simulink model "Commander_Stabilizer_QDrone"  (R2021b)
settings: Solver=ode1  StartTime=0.0  StopTime=inf  FixedStep=0.001  RelTol=1e-3  EnableMultiTasking=on
InitFcn:
  | set_param(gcs, 'ZoomFactor','FitSystem')
model workspace (MAT data in the model file):
  target_system = 1
undefined symbols (not defined in the file): HIL, qc_get_step_size
libraries: quarc_library x49, simulink x23, simulink_extras x5
(part 3 of 3)

== system Commander_Stabilizer_QDrone/PHYSICAL PLANT w// LINEAR THRUST/Sensor Failure Monitoring/Sensor Failure (Accelerometer) ==
  note: Check for flat-line ZERO Accelerometer data (no data)
  Sensor Input : Inport
  Clock : Clock
  Compare To Constant : simulink/Logic and Bit Operations/Compare To Constant  relop=>=  const=1  OutDataTypeStr=boolean
  Demux1 : Demux  Outputs=3
  Logical Operator : Logic  Operator=OR  Inputs=3  AllPortsSameDT=off  OutDataTypeStr=boolean
  Logical Operator1 : Logic  AllPortsSameDT=off  OutDataTypeStr=boolean
  Terminator1 : Terminator
  Terminator3 : Terminator
  Terminator4 : Terminator
  Threshold : quarc_library/Discontinuities/Threshold  operator===  param_src=Specify via dialog  threshold=0  duration=1
      settings: SourceProductName=The database C:\Users\user\AppData\Roaming\MathWorks\MATLAB\R2017a\slblocks_master.db is locked, or a table in the database is locked. (database is locked)
  Threshold1 : quarc_library/Discontinuities/Threshold  operator===  param_src=Specify via dialog  threshold=0  duration=1
      settings: SourceProductName=The database C:\Users\user\AppData\Roaming\MathWorks\MATLAB\R2017a\slblocks_master.db is locked, or a table in the database is locked. (database is locked)
  Threshold2 : quarc_library/Discontinuities/Threshold  operator===  param_src=Specify via dialog  threshold=0  duration=1
      settings: SourceProductName=The database C:\Users\user\AppData\Roaming\MathWorks\MATLAB\R2017a\slblocks_master.db is locked, or a table in the database is locked. (database is locked)
  Sensor Fault : Outport  VectorParamsAs1DForOutWhenUnconnected=off
  wires:
  Threshold/2 -> Terminator1/1
  Threshold1/2 -> Terminator3/1
  Logical Operator/1 -> Logical Operator1/2
  Demux1/2 -> Threshold1/1
  Demux1/3 -> Threshold2/1
  Demux1/1 -> Threshold/1
  Threshold2/1 -> Logical Operator/3
  Threshold2/2 -> Terminator4/1
  Sensor Input/1 -> Demux1/1
  Logical Operator1/1 -> Sensor Fault/1
  Compare To Constant/1 -> Logical Operator1/1
  Threshold1/1 -> Logical Operator/2
  Threshold/1 -> Logical Operator/1
  Clock/1 -> Compare To Constant/1

== system Commander_Stabilizer_QDrone/PHYSICAL PLANT w// LINEAR THRUST/Sensor Failure Monitoring/Sensor Failure (Gyroscope) ==
  note: Check for flat-line ZERO Gyro data (no data)
  Sensor Input : Inport
  Clock : Clock
  Compare To Constant : simulink/Logic and Bit Operations/Compare To Constant  relop=>=  const=1  OutDataTypeStr=boolean
  Demux1 : Demux  Outputs=3
  Logical Operator : Logic  Operator=OR  Inputs=3  AllPortsSameDT=off  OutDataTypeStr=boolean
  Logical Operator1 : Logic  AllPortsSameDT=off  OutDataTypeStr=boolean
  Terminator1 : Terminator
  Terminator3 : Terminator
  Terminator4 : Terminator
  Threshold : quarc_library/Discontinuities/Threshold  operator===  param_src=Specify via dialog  threshold=0  duration=1
      settings: SourceProductName=The database C:\Users\user\AppData\Roaming\MathWorks\MATLAB\R2017a\slblocks_master.db is locked, or a table in the database is locked. (database is locked)
  Threshold1 : quarc_library/Discontinuities/Threshold  operator===  param_src=Specify via dialog  threshold=0  duration=1
      settings: SourceProductName=The database C:\Users\user\AppData\Roaming\MathWorks\MATLAB\R2017a\slblocks_master.db is locked, or a table in the database is locked. (database is locked)
  Threshold2 : quarc_library/Discontinuities/Threshold  operator===  param_src=Specify via dialog  threshold=0  duration=1
      settings: SourceProductName=The database C:\Users\user\AppData\Roaming\MathWorks\MATLAB\R2017a\slblocks_master.db is locked, or a table in the database is locked. (database is locked)
  Sensor Fault : Outport  VectorParamsAs1DForOutWhenUnconnected=off
  wires:
  Clock/1 -> Compare To Constant/1
  Threshold/1 -> Logical Operator/1
  Threshold1/1 -> Logical Operator/2
  Compare To Constant/1 -> Logical Operator1/1
  Logical Operator1/1 -> Sensor Fault/1
  Sensor Input/1 -> Demux1/1
  Threshold2/2 -> Terminator4/1
  Threshold2/1 -> Logical Operator/3
  Demux1/1 -> Threshold/1
  Demux1/3 -> Threshold2/1
  Demux1/2 -> Threshold1/1
  Logical Operator/1 -> Logical Operator1/2
  Threshold1/2 -> Terminator3/1
  Threshold/2 -> Terminator1/1

== matlab function Commander_Stabilizer_QDrone/HORIZON FRAME CONVERSION AND ESTIMATION/Pose Switchbox/MATLAB Function4 ==
  data: sigmoid_type input; enable output; yaw_des input; slow_lim input; fast_lim input; yaw_cur input; yaw_ref output; max_yaw_vel output; max_yaw_accel output; yaw_vel input
function [enable, yaw_ref, max_yaw_vel, max_yaw_accel] = fcn(sigmoid_type, yaw_des, slow_lim, fast_lim, yaw_cur, yaw_vel)

% Note: Some of the cases below are identical. However, they are separated out 
% based on the states of the state machine for ease of modification in the future. 
% For example, states 4 and 5 are identical. However, if the user wants different 
% signmoid behaviour when taking off than when landing, these cases may not be the same. 

enable = 0;
yaw_ref = 0;
max_yaw_vel = 0;
max_yaw_accel = 0;

switch sigmoid_type
    case 1 % This is for the IDLE, ARM, E_ABORT, E_STOP and DISABLE states of the FSM
        enable = 0;
        yaw_ref = 0;
        max_yaw_vel = 0;
        max_yaw_accel = 0;
    case 2 % This is for the TAKEOFF THROTTLE state of the FSM
        enable = 1;
        yaw_ref = yaw_des;
        max_yaw_vel = slow_lim(1);
        max_yaw_accel = slow_lim(2);  
    case 3 % This is for the FLIGHT state of the FSM 
        enable = 1;
        yaw_ref = yaw_des;
        max_yaw_vel = fast_lim(1);
        max_yaw_accel = fast_lim(2);
    case 4 % This is for the TAKEOFF HEIGHT state of the FSM
        enable = 1;
        yaw_ref = yaw_des;
        if (yaw_vel < 0)||(yaw_des < yaw_cur)||(abs(yaw_cur-yaw_des)<=0.2)
            max_yaw_vel = fast_lim(1);
            max_yaw_accel = fast_lim(2);
        else    
            max_yaw_vel = slow_lim(1);
            max_yaw_accel = slow_lim(2);
        end
    case 5 % This is for the AUTOLAND state of the FSM
        enable = 1;
        yaw_ref = yaw_des;
        if (yaw_vel >= 0)
            max_yaw_vel = fast_lim(1);
            max_yaw_accel = fast_lim(2);
        else    
            max_yaw_vel = slow_lim(1);
            max_yaw_accel = slow_lim(2);
        end
end

== matlab function Commander_Stabilizer_QDrone/HORIZON FRAME CONVERSION AND ESTIMATION/Pose Switchbox/Signmoid Type ==
  data: FSM_state input; sigmoid_type output
function sigmoid_type  = sigmoid_type_position(FSM_state)

% QDrone: Position Switchbox
%
% Switching between different sigmoid types based on 
% which state the FSM is in.
%
% v3.0 - 4th October, 2018
%
% INPUTS:
% -------
% FSM_state = current state of the FSM------------------------------------------------------- (#)         [1]
% 
% OUTPUTS:
% --------
% sigmoid_type = an integer whose state determines how the commands/measurements are transformed-- (#)         [1]

% Sigmoid_type = 1; This is for the IDLE, ARM, E_ABORT, E_STOP and DISABLE states of the FSM
% Sigmoid_type = 2; This is for the TAKEOFF THROTTLE state of the FSM
% Sigmoid_type = 3; This is for the FLIGHT state of the FSM
% Sigmoid_type = 4; This is for the TAKEOFF HEIGHT state of the FSM
% Sigmoid_type = 5; This is for the AUTOLAND state of the FSM

sigmoid_type = 0;

switch FSM_state
    case 1 % IDLE STATE
        sigmoid_type = 1;
    case 2 % ARM STATE
        sigmoid_type = 1;
    case 3 % TAKEOFF THROTTLE STATE
        sigmoid_type = 2;
    case 4 % TAKEOFF HEIGHT STATE
        sigmoid_type = 4;
    case 5 % FLIGHT STATE
        sigmoid_type = 3;
    case 6 % AUTOLAND STATE
        sigmoid_type = 5;
    case 7 % EMERGENCY STOP STATE
        sigmoid_type = 1;
    case 8 % EMERGENCY ABORT STATE
        sigmoid_type = 1;
    case 9 % DISABLE STATE
        sigmoid_type = 1;
end

== matlab function Commander_Stabilizer_QDrone/COMMANDER (ANGLE MODE)/THROTTLE SWITCHBOX /Hover Throttle Sigmoid Parameters ==
  data: sigmoid_type input; enable output; trim_throttle input; takeoff_lim input; land_lim input; throttle_vel input; throttle_ref output; max_throttle_vel output; max_throttle_accel output
function [enable, throttle_ref, max_throttle_vel, max_throttle_accel] = fcn(sigmoid_type, trim_throttle, takeoff_lim, land_lim, throttle_vel)

% Note: Some of the cases below are identical. However, they are separated out 
% based on the states of the state machine for ease of modification in the future. 
% For example, states 4 and 5 are identical. However, if the user wants different 
% signmoid behaviour when taking off than when landing, these cases may not be the same. 

enable = 0;
throttle_ref = 0;
max_throttle_vel = 0;
max_throttle_accel = 0;

switch sigmoid_type
    case 1 % sigmoid = 1 - Command 0 throttle
        % This is for the IDLE, ARM, E_ABORT, and DISABLE states of the FSM
        enable = 0;
        throttle_ref = 0;
        max_throttle_vel = 0;
        max_throttle_accel = 0;

    case 2 % sigmoid = 2 - Sigmoid throttle up from 0 to the trim value
        % This is for the TAKEOFF THROTTLE state of the FSM
        enable = 1;
        throttle_ref = trim_throttle;
        max_throttle_vel = takeoff_lim(1);
        max_throttle_accel = takeoff_lim(2);

    case 3 % sigmoid = 3 - Pass controller throttle straight through + trim value.
        % This is for the TAKEOFF HEIGHT and FLIGHT state of the FSM
        enable = 1;
        throttle_ref = trim_throttle;
        max_throttle_vel = takeoff_lim(1);
        max_throttle_accel = takeoff_lim(2);

    case 4 % sigmoid = 4 - Ignore controller throttle. Sigmoid it down to 0.
        % This is for the E_Landing state of the FSM
        enable = 1;
        throttle_ref = 0;
        if throttle_vel > 0
            max_throttle_vel = takeoff_lim(1);
            max_throttle_accel = takeoff_lim(2);
        else
            max_throttle_vel = land_lim(1);
            max_throttle_accel = land_lim(2);
        end
        
    case 5 % sigmoid = 5 - Pass controller throttle straight through + trim value.
        % This is for the AUTOLAND state of the FSM
        enable = 1;
        throttle_ref = trim_throttle;
        max_throttle_vel = takeoff_lim(1);
        max_throttle_accel = takeoff_lim(2);

end

== matlab function Commander_Stabilizer_QDrone/COMMANDER (ANGLE MODE)/STATE MACHINE LOGIC ==
  data: E_Abort output; isArm output; pt_ARM_to_TAKEOFF_THROTTLE output; pt_TAKE_OFF_HEIGHT_TO_AUTOLAND output; pt_FLIGHT_TO_AUTOLAND output; current_state input; initializing input; Tracking_Issue input; Communication_Issue input; low_battery input; trigger_1 input; trigger_2 input; E_abort input; joystick_issue input; net_throttle_at_trim input; net_throttle_close_to_zero input; ctrl_throttle_close_to_zero input; take_off_successful input; flying_too_low input; flying_too_high input; close_to_ground input; pt_TAKEOFF_THROTTLE_TO_TAKEOFF_HEIGHT output; pt_TAKE_OFF_HEIGHT_TO_FLIGHT output; pt_AUTOLAND_TO_DISABLE output; pt_EMERGENCY_STOP_TO_DISABLE output; pt_EMERGENCY_ABORT_TO_DISABLE output; Error output; stop_model output; sensor_failed input
function [E_Abort, isArm, pt_ARM_to_TAKEOFF_THROTTLE, pt_TAKE_OFF_HEIGHT_TO_AUTOLAND, pt_FLIGHT_TO_AUTOLAND, pt_TAKEOFF_THROTTLE_TO_TAKEOFF_HEIGHT, pt_TAKE_OFF_HEIGHT_TO_FLIGHT, pt_AUTOLAND_TO_DISABLE, pt_EMERGENCY_STOP_TO_DISABLE, pt_EMERGENCY_ABORT_TO_DISABLE, Error, stop_model]...
    = SM_logic(current_state, initializing, Tracking_Issue, Communication_Issue, low_battery, trigger_1, trigger_2, E_abort, joystick_issue,...
    net_throttle_at_trim, net_throttle_close_to_zero, ctrl_throttle_close_to_zero, take_off_successful, flying_too_low, flying_too_high, close_to_ground, sensor_failed)

% Programmatic Logic Block
%
% Logic for the FSM is generated here based on a variety of signals.
% Mostly, logic to programmatically trigger the transition to either a 
% natural next state, or an Error state, is generated here.
%
% Last modified: March, 2020
%
% INPUTS:
% -------
% current_state = previous state of the FSM-------------------------------------------------- (#)         [1]
% initializing = signal representing that the system is initializing (first 5s + buffer)- - - (bool)      [1]
% comm = communication signal representing MAVLINK connection-------------------------------- (bool)      [1]
% peripheral = signal representing joystick and optitrack connection- - - - - - - - - - - - - (bool)      [2]
% low_battery = signal representing low battery---------------------------------------------- (bool)      [1]
% trigger_1 = trigger representing ARM/DISARM - - - - - - - - - - - - - - - - - - - - - - - - (bool)      [1]
% trigger_2 = trigger representing TAKEOFF/AUTOLAND------------------------------------------ (bool)      [1]
% motors_not_spinning = signal representing the motors not spinning - - - - - - - - - - - - - (bool)      [1]
% net_throttle_at_trim = trim throttle for the application drone ---------------------------- (bool)      [1]
% net_throttle_close_to_zero = net throttle is close to zero in emergency stop mode - - - - - (bool)      [1]
% ctrl_throttle_close_to_zero = ctrl throttle is close to zero in emergency stop mode - - - - (bool)      [1]
% take_off_successful = signal representing whether drone has taken-off successfully -------- (bool)      [1]
% flying_too_low = signal representing whether the drone's height is below threshold and cmd- (bool)      [1]
% flying_too_high = signal representing whether the drone's height is above threshold-------- (bool)      [1]
% close_to_ground = signal representing whether the drone is close to the ground to autoland- (bool)      [1]
% 
% OUTPUTS:
% --------
% Error = Whether an Error is issued or not                                                             (bool)    [1]
% E_Abort = fed through for ease of understanding flow (see STATE MACHINE TRANSITION BLOCK)             (bool)    [1]
% isArm = programmatic transition state                                                                 (bool)    [1]
% pt_ARM_to_TAKEOFF_THROTTLE = programmatic transition state BEGIN_STATE_TO_FINAL_STATE                 (bool)    [1]
% pt_TAKEOFF_THROTTLE_TO_TAKEOFF_HEIGHT = programmatic transition state BEGIN_STATE_TO_FINAL_STATE      (bool)    [1]
% pt_TAKE_OFF_HEIGHT_TO_AUTOLAND = programmatic transition state BEGIN_STATE_TO_FINAL_STATE             (bool)    [1]
% pt_TAKEOFF_THROTTLE_TO_TAKEOFF_HEIGHT = programmatic transition state BEGIN_STATE_TO_FINAL_STATE      (bool)    [1]
% pt_TAKE_OFF_HEIGHT_TO_FLIGHT = programmatic transition state BEGIN_STATE_TO_FINAL_STATE               (bool)    [1]
% pt_AUTOLAND_TO_DISABLE = programmatic transition state BEGIN_STATE_TO_FINAL_STATE                     (bool)    [1]
% pt_EMERGENCY_STOP_TO_DISABLE = programmatic transition state BEGIN_STATE_TO_FINAL_STATE               (bool)    [1]
% pt_EMERGENCY_ABORT_TO_DISABLE = programmatic transition state BEGIN_STATE_TO_FINAL_STATE              (bool)    [1]
% stop_model = STOP THE MODEL AFTER                                                                     (bool)    [1]

Error = 0;
E_Abort = E_abort;
isArm = false;
pt_ARM_to_TAKEOFF_THROTTLE = false;
pt_TAKEOFF_THROTTLE_TO_TAKEOFF_HEIGHT = false;
pt_TAKE_OFF_HEIGHT_TO_AUTOLAND = false;
pt_TAKE_OFF_HEIGHT_TO_FLIGHT = false;
pt_FLIGHT_TO_AUTOLAND = false;
pt_AUTOLAND_TO_DISABLE = false;
pt_EMERGENCY_STOP_TO_DISABLE = false;
pt_EMERGENCY_ABORT_TO_DISABLE = false;
stop_model = 0;

switch current_state
    %---------------------------------------------------------------------%
    case 1 % IDLE STATE
        if (Communication_Issue)||...          % Communication issue
           (joystick_issue)||...               % joystick issue
           (Tracking_Issue)||...               % optitrack issue
           (low_battery)||...                  % low batter  
           (sensor_failed)||...                % if sensor (IMU) failure is detected on drone stabilizer    
           ((trigger_1)&&(initializing))||...  % armed while initializing
           (trigger_2)&&(initializing)||...    % tried to takeoff while initializing
           (~ctrl_throttle_close_to_zero)      % if throttle isn't at zero, don't arm
           %----------------------------------------%
            Error = 1;
        elseif trigger_1 % user arms
            isArm = true;
        end
    %---------------------------------------------------------------------%    
    case 2 % ARMED STATE
        isArm = trigger_1;
        if (Communication_Issue)||...          % Communication issue
           (joystick_issue)||...               % joystick issue
           (Tracking_Issue)||...               % optitrack issue
           (low_battery)||...                  % low battery
           (sensor_failed)||...                % if sensor (IMU) failure is detected on drone stabilizer
           (~ctrl_throttle_close_to_zero)      % if throttle isn't at zero, don't arm
           %----------------------------------------%
            Error = 1;
        elseif trigger_1 && trigger_2
            pt_ARM_to_TAKEOFF_THROTTLE = true;
        end        
    %---------------------------------------------------------------------%
    case 3 % TAKEOFF_THROTTLE STATE
        if (Communication_Issue)||...     % Communication issue
           (joystick_issue)||...          % joystick issue
           (Tracking_Issue)||...          % optitrack issue           
           (low_battery)||...             % low battery
           (sensor_failed)||...           % if sensor (IMU) failure is detected on drone stabilizer
           (~trigger_1)||...              % user disarms
           (~trigger_2)||...              % user commands auto-land before drone starts taking off
           (~ctrl_throttle_close_to_zero) % if throttle isn't at zero, don't arm
           %----------------------------------------%
            Error = 1;
        elseif (joystick_issue)           % joystick issue
            pt_TAKE_OFF_HEIGHT_TO_AUTOLAND = true;
        elseif net_throttle_at_trim
            pt_TAKEOFF_THROTTLE_TO_TAKEOFF_HEIGHT = true;
        end
    %---------------------------------------------------------------------%
    case 4 % TAKEOFF_HEIGHT STATE
        if (Communication_Issue)||... % Communication issue
           (joystick_issue)||...      % joystick issue
           (Tracking_Issue)||...      % optitrack issue
           (sensor_failed)||...       % if sensor (IMU) failure is detected on drone stabilizer    
           (flying_too_low)||...      % current height is below safety threshold 
           (flying_too_high)||...     % flying above safety margin (w.r.t optitrack)
           (~trigger_1)               % user disarms
            %----------------------------------------%
            Error = 1;
        elseif (~trigger_2)||low_battery 
            pt_TAKE_OFF_HEIGHT_TO_AUTOLAND = true;
        elseif take_off_successful
            pt_TAKE_OFF_HEIGHT_TO_FLIGHT = true;
        end
    %---------------------------------------------------------------------%
    case 5 % FLIGHT STATE
        if (Communication_Issue)||...   % Communication issue
           (joystick_issue)||...        % joystick issue
           (Tracking_Issue)||...        % optitrack issue
           (sensor_failed)||...         % if sensor (IMU) failure is detected on drone stabilizer
           (flying_too_low)||...        % current height is below safety threshold  
           (flying_too_high)||...       % flying above safety margin (w.r.t optitrack)
           (~trigger_1)                 % user disarms
           %----------------------------------------%
            Error = 1;
        elseif (~trigger_2)||low_battery
            pt_FLIGHT_TO_AUTOLAND = true;
        end
    %---------------------------------------------------------------------%
    case 6 % AUTOLAND STATE
        if (Communication_Issue)||...  % Communication issue
           (joystick_issue)||...       % joystick issue
           (Tracking_Issue)||...       % optitrack issue
           (sensor_failed)||...        % if sensor (IMU) failure is detected on drone stabilizer
           (flying_too_high)||...      % flying above safety margin (w.r.t optitrack)    
           (~trigger_1)||...           % user disarms
           (trigger_2)                 % user tries to takeoff while landing
           
           
           %----------------------------------------%
            Error = 1;
        elseif close_to_ground 
            pt_AUTOLAND_TO_DISABLE = true;
        end
    %---------------------------------------------------------------------%
    case 7 % EMERGENCY LAND STATE
        if net_throttle_close_to_zero 
            pt_EMERGENCY_STOP_TO_DISABLE = true;
        end
    %---------------------------------------------------------------------%
    case 8 % EMERGENCY ABORT STATE
        pt_EMERGENCY_ABORT_TO_DISABLE = true;
    %---------------------------------------------------------------------%
    case 9
        % Stop the model.
        stop_model = 1;
end

== matlab function Commander_Stabilizer_QDrone/PHYSICAL PLANT w// LINEAR THRUST/Red - Low Voltage Green - Armed Blue - Disarmed/MATLAB Function LED Color Assignment ==
  data: arm input; value output; low_battery input
function value = fcn(arm, low_battery)

if low_battery
    value = 1;
elseif arm
    value = 2;
else 
    value = 3;
end

== matlab function Commander_Stabilizer_QDrone/COMMANDER (ANGLE MODE)/STATE MACHINE TRANSITION ==
  data: current_state input; E_Abort input; isArm input; pt_ARM_to_TAKEOFF_THROTTLE input; pt_TAKE_OFF_HEIGHT_TO_AUTOLAND input; pt_FLIGHT_TO_AUTOLAND input; Next_state output; pt_TAKEOFF_THROTTLE_TO_TAKEOFF_HEIGHT input; pt_TAKE_OFF_HEIGHT_TO_FLIGHT input; pt_AUTOLAND_TO_DISABLE input; pt_EMERGENCY_STOP_TO_DISABLE input; pt_EMERGENCY_ABORT_TO_DISABLE input; Error input
function Next_state = SM_transition(current_state, E_Abort, isArm, pt_ARM_to_TAKEOFF_THROTTLE, pt_TAKE_OFF_HEIGHT_TO_AUTOLAND, pt_FLIGHT_TO_AUTOLAND, pt_TAKEOFF_THROTTLE_TO_TAKEOFF_HEIGHT, pt_TAKE_OFF_HEIGHT_TO_FLIGHT, pt_AUTOLAND_TO_DISABLE, pt_EMERGENCY_STOP_TO_DISABLE, pt_EMERGENCY_ABORT_TO_DISABLE, Error)

% Programmatic Transition Block
%
% FINITE STATE MACHINE (FSM) with 9 states as described below, transitioning based on the 
% values of the isArm, transition signals, Error, and E_Abort
%
% Last modified: March, 2020
%
% INPUTS:
% ------
% current_state = Current state of the FSM        (#)     [1]
% E_Abort                                         (bool)  [1]
% isArm                                           (bool)  [1]
% pt_ARM_TO_TAKEOFF_THROTTLE                      (bool)  [1]
% pt_TAKE_OFF_HEIGHT_TO_AUTOLAND                  (bool)  [1]
% pt_FLIGHT_TO_AUTOLAND                           (bool)  [1]
% pt_TAKEOFF_THROTTLE_TO_TAKEOFF_HEIGHT           (bool)  [1]
% pt_TAKE_OFF_HEIGHT_TO_FLIGHT                    (bool)  [1]
% pt_AUTOLAND_TO_DISABLE                          (bool)  [1]
% pt_EMERGENCY_STOP_TO_DISABLE                    (bool)  [1]
% pt_EMERGENCY_ABORT_TO_DISABLE                   (bool)  [1]
% Error                                           (bool)  [1]
%
% OUTPUT:
% -------
% Next_state = Next state of the FSM              (#)     [1]

Next_state = double(0);
switch current_state
%-------------------------------------------------------------------------%
    case 1 % IDLE STATE
        if E_Abort
            Next_state = 8; % GOTO EMERGENCY ABORT STATE
        elseif Error
            Next_state = 7; % GOTO EMERGENCY STOP STATE
        elseif isArm
            Next_state = 2; % GOTO ARMED STATE
        else
            Next_state = 1; % STAY IN IDLE STATE
        end
%-------------------------------------------------------------------------%
    case 2 % ARMED STATE
        if E_Abort
            Next_state = 8; % GOTO EMERGENCY ABORT STATE
        elseif Error
            Next_state = 7; % GOTO EMERGENCY STOP STATE
        elseif ~isArm
            Next_state = 1; % GOTO IDLE STATE
        elseif pt_ARM_to_TAKEOFF_THROTTLE
            Next_state = 3; % GOTO TAKEOFF_THROTTLE STATE 
        else
            Next_state = 2; % STAY IN ARMED STATE
        end
%-------------------------------------------------------------------------%
    case 3 % TAKEOFF_THROTTLE STATE
        if E_Abort
            Next_state = 8; % GOTO EMERGENCY ABORT STATE
        elseif Error
            Next_state = 7; % GOTO EMERGENCY STOP STATE
        elseif pt_TAKEOFF_THROTTLE_TO_TAKEOFF_HEIGHT
            Next_state = 4; % GOTO TAKEOFF_HEIGHT STATE
        else
            Next_state = 3; % STAY IN TAKEOFF_THROTTLE STATE
        end
%-------------------------------------------------------------------------%
    case 4 % TAKEOFF_HEIGHT STATE
        if E_Abort
            Next_state = 8; % GOTO EMERGENCY ABORT STATE
        elseif Error
            Next_state = 7; % GOTO EMERGENCY STOP STATE
        elseif pt_TAKE_OFF_HEIGHT_TO_AUTOLAND
            Next_state = 6;
        elseif pt_TAKE_OFF_HEIGHT_TO_FLIGHT
            Next_state = 5; % GOTO FLIGHT STATE
        else
            Next_state = 4; % STAY IN TAKEOFF_HEIGHT STATE
        end
%-------------------------------------------------------------------------%
    case 5 % FLIGHT STATE
        if E_Abort
            Next_state = 8; % GOTO EMERGENCY ABORT STATE
        elseif Error
            Next_state = 7; % GOTO EMERGENCY STOP STATE
        elseif pt_FLIGHT_TO_AUTOLAND
            Next_state = 6; % GOTO AUTO_LAND STATE
        else
            Next_state = 5; % STAY IN FLIGHT STATE
        end
%-------------------------------------------------------------------------%       
    case 6 % AUTO_LAND STATE
        if E_Abort
            Next_state = 8; % GOTO EMERGENCY ABORT STATE
        elseif Error
            Next_state = 7; % GOTO EMERGENCY STOP STATE
        elseif pt_AUTOLAND_TO_DISABLE
            Next_state = 9; % GOTO DISABLE STATE
        else
            Next_state = 6; % STAY IN AUTO_LAND STATE
        end
%-------------------------------------------------------------------------%
    case 7 % EMERGENCY STOP STATE
        if E_Abort
            Next_state = 8; % GOTO EMERGENCY ABORT STATE
        elseif pt_EMERGENCY_STOP_TO_DISABLE
            Next_state = 9; % GOTO DISABLE STATE
        else
            Next_state = 7; % STAY IN EMERGENCY STOP STATE
        end
%-------------------------------------------------------------------------%
    case 8 % EMERGENCY ABORT
        if pt_EMERGENCY_ABORT_TO_DISABLE
            Next_state = 9; % GOTO DISABLE STATE
        else 
            Next_state = 8; % STAY IN EMERGENCY ABORT STATE
        end
%-------------------------------------------------------------------------%    
    case 9 % DISABLE
        Next_state = 9; % Always stay in DISABLE state if you are here    
end

== matlab function Commander_Stabilizer_QDrone/Communication/Detect Communication Loss/MATLAB Function ==
  settings: updateMethod=DISCRETE
  data: time input; stream_connection_loss output; state input; error input; ms_time input; data_loss output
function [stream_connection_loss , data_loss] = fcn(time, state, error, ms_time)

persistent ms_time_prev
    if isempty(ms_time_prev)
        ms_time_prev = 0;
    end

stream_connection_loss = 0;
data_loss = 0;
if time > 3
    if ((state ~= 2)&&(error < 0))
        % stream connection is not established correctly
        stream_connection_loss = 1;
    end

    if (ms_time == ms_time_prev)&&(ms_time > 0)
        % data is stale
        data_loss = 1;
    end
end

ms_time_prev = ms_time;

== matlab function Commander_Stabilizer_QDrone/PHYSICAL PLANT w// LINEAR THRUST/roll and pitch approximation from accelerometer ==
  data: roll_acc output; pitch_acc output; acc_body input
function [roll_acc, pitch_acc]   = fcn(acc_body)
%#eml
n = norm(acc_body,2);
if n>eps
    acc_body = acc_body/n; 
else
    acc_body = [0 0 1]';
end

roll_acc = atan2(acc_body(2),acc_body(3));
pitch_acc = atan2( -acc_body(1), acc_body(2)*sin(roll_acc)+acc_body(3)*cos(roll_acc));

== matlab function Commander_Stabilizer_QDrone/COMMANDER (ANGLE MODE)/THROTTLE SWITCHBOX /Throttle Switchbox ==
  data: FSM_state input; sigmoid output
function sigmoid  = application_drone_throttle_switchbox(FSM_state)

% Application Drone: Throttle Switchbox
%
% Logic for switching between throttle commands from the controller 
%
% v2.0 - 5th october, 2018
%
% INPUTS:
% -------
% FSM_state = current state of the FSM------------------------------------------------------- (#)         [1]
% 
% OUTPUTS:
% --------
% sigmoid = an integer whose state determines how the heights are transformed---------------- (#)         [1]
% sigmoid = 1 - Command 0 throttle
% sigmoid = 2 - Sigmoid throttle up from 0 to the trim value
% sigmoid = 3 - Pass controller throttle straight through + trim value.
% sigmoid = 4 - Ignore controller throttle. Sigmoid it down to 0.
% sigmoid = 5 - Pass controller throttle straight through + trim value.


sigmoid = 0;
switch FSM_state
    case 1 % IDLE STATE
        sigmoid = 1;
    case 2 % ARM STATE
        sigmoid = 1;
    case 3 % TAKEOFF THROTTLE STATE
        sigmoid = 2;
    case 4 % TAKEOFF HEIGHT STATE
        sigmoid = 3;
    case 5 % FLIGHT STATE
        sigmoid = 3;
    case 6 % AUTOLAND STATE
        sigmoid = 5;
    case 7 % EMERGENCY STOP STATE
        sigmoid = 4;
    case 8 % EMERGENCY ABORT STATE
        sigmoid = 1;
    case 9 % DISABLE STATE
        sigmoid = 1;
end

== matlab function Commander_Stabilizer_QDrone/HORIZON FRAME CONVERSION AND ESTIMATION/Pose Switchbox/MATLAB Function ==
  data: sigmoid_type input; enable output; x_des input; slow_lim input; fast_lim input; x_cur input; x_vel input; x_ref output; max_x_vel output; max_x_accel output; x_meas input
function [enable, x_ref, max_x_vel, max_x_accel] = fcn(sigmoid_type, x_des, slow_lim, fast_lim, x_cur, x_vel, x_meas)

% Note: Some of the cases below are identical. However, they are separated out 
% based on the states of the state machine for ease of modification in the future. 
% For example, states 4 and 5 are identical. However, if the user wants different 
% signmoid behaviour when taking off than when landing, these cases may not be the same. 

enable = 0;
x_ref = 0;
max_x_vel = 0;
max_x_accel = 0;

switch sigmoid_type
    case 1 % This is for the IDLE, ARM, E_ABORT, E_STOP and DISABLE states of the FSM
        enable = 1;
        x_ref = x_meas;
        max_x_vel = slow_lim(1);
        max_x_accel = slow_lim(2);

    case 2 % This is for the TAKEOFF THROTTLE state of the FSM
        enable = 1;
        x_ref = x_meas;
        max_x_vel = slow_lim(1);
        max_x_accel = slow_lim(2);

    case 3 % This is for the FLIGHT state of the FSM
        enable = 1;
        x_ref = x_des;
        max_x_vel = fast_lim(1);
        max_x_accel = fast_lim(2);

    case 4 % This is for the TAKEOFF HEIGHT state of the FSM
        enable = 1;
        x_ref = x_des;
        if (abs(x_cur - x_des) <= 0.02)
            max_x_vel = fast_lim(1);
            max_x_accel = fast_lim(2);
        else    
            max_x_vel = slow_lim(1);
            max_x_accel = slow_lim(2);
        end
    case 5 % This is for the AUTOLAND state of the FSM
        enable = 1;
        x_ref = x_des;
        if (abs(x_cur - x_des) <= 0.02)
            max_x_vel = fast_lim(1);
            max_x_accel = fast_lim(2);        
        else
            max_x_vel = slow_lim(1);
            max_x_accel = slow_lim(2);
        end
        
end

== matlab function Commander_Stabilizer_QDrone/HORIZON FRAME CONVERSION AND ESTIMATION/Pose Switchbox/MATLAB Function1 ==
  data: sigmoid_type input; enable output; y_des input; slow_lim input; fast_lim input; y_cur input; y_vel input; y_ref output; max_y_vel output; max_y_accel output; y_meas input
function [enable, y_ref, max_y_vel, max_y_accel] = fcn(sigmoid_type, y_des, slow_lim, fast_lim, y_cur, y_vel, y_meas)

% Note: Some of the cases below are identical. However, they are separated out 
% based on the states of the state machine for ease of modification in the future. 
% For example, states 4 and 5 are identical. However, if the user wants different 
% signmoid behaviour when taking off than when landing, these cases may not be the same. 

enable = 0;
y_ref = 0;
max_y_vel = 0;
max_y_accel = 0;

switch sigmoid_type
    case 1 % This is for the IDLE, ARM, E_ABORT, E_STOP and DISABLE states of the FSM
        enable = 1;
        y_ref = y_meas;
        max_y_vel = slow_lim(1);
        max_y_accel = slow_lim(2);

    case 2 % This is for the TAKEOFF THROTTLE state of the FSM
        enable = 1;
        y_ref = y_meas;
        max_y_vel = slow_lim(1);
        max_y_accel = slow_lim(2);

    case 3 % This is for the FLIGHT state of the FSM
        enable = 1;
        y_ref = y_des;
        max_y_vel = fast_lim(1);
        max_y_accel = fast_lim(2);

    case 4 % This is for the TAKEOFF HEIGHT state of the FSM
        enable = 1;
        y_ref = y_des;
        if (abs(y_cur - y_des) <= 0.02)
            max_y_vel = fast_lim(1);
            max_y_accel = fast_lim(2);
        else    
            max_y_vel = slow_lim(1);
            max_y_accel = slow_lim(2);
        end
    case 5 % This is for the AUTOLAND state of the FSM
        enable = 1;
        y_ref = y_des;
        if (abs(y_cur - y_des) <= 0.02)
            max_y_vel = fast_lim(1);
            max_y_accel = fast_lim(2);        
        else
            max_y_vel = slow_lim(1);
            max_y_accel = slow_lim(2);
        end
        
end

== matlab function Commander_Stabilizer_QDrone/HORIZON FRAME CONVERSION AND ESTIMATION/Pose Switchbox/MATLAB Function2 ==
  data: sigmoid_type input; enable output; height_des input; slow_lim input; fast_lim input; height_cur input; height_vel input; height_ref output; max_height_vel output; max_height_accel output
function [enable, height_ref, max_height_vel, max_height_accel] = fcn(sigmoid_type, height_des, slow_lim, fast_lim, height_cur, height_vel)

% Note: Some of the cases below are identical. However, they are separated out 
% based on the states of the state machine for ease of modification in the future. 
% For example, states 4 and 5 are identical. However, if the user wants different 
% signmoid behaviour when taking off than when landing, these cases may not be the same. 

enable = 0;
height_ref = 0;
max_height_vel = 0;
max_height_accel = 0;

switch sigmoid_type
    case 1 % This is for the IDLE, ARM, E_ABORT, E_STOP and DISABLE states of the FSM
        enable = 0;
        height_ref = 0;
        max_height_vel = 0;
        max_height_accel = 0;

    case 2 % This is for the TAKEOFF THROTTLE state of the FSM
        enable = 0;
        height_ref = 0;
        max_height_vel = 0;
        max_height_accel = 0;

    case 3 % This is for the FLIGHT state of the FSM 
        enable = 1;
        height_ref = height_des;
        max_height_vel = fast_lim(1);
        max_height_accel = fast_lim(2);

    case 4 % This is for the TAKEOFF HEIGHT state of the FSM
        enable = 1;
        height_ref = height_des;
        if (height_vel < 0)||(abs(height_cur - height_des) <= 0.1)||(height_des <= height_cur)
            max_height_vel = fast_lim(1);
            max_height_accel = fast_lim(2);
        else    
            max_height_vel = slow_lim(1);
            max_height_accel = slow_lim(2);
        end
    case 5 % This is for the AUTOLAND state of the FSM
        enable = 1;
        height_ref = 0;
        if height_vel >= 0
            max_height_vel = fast_lim(1);
            max_height_accel = fast_lim(2);        
        else
            max_height_vel = slow_lim(1);
            max_height_accel = slow_lim(2);
        end
        
end
